simulink model "Partie4_Registre"  (R2026b)
settings: Solver=FixedStepDiscrete  StopTime=65*Tb  FixedStep=Tb
undefined symbols (not defined in the file): Tb
settings Model: Creator=WORLD COMPUTERS  LastModifiedBy=WORLD COMPUTERS

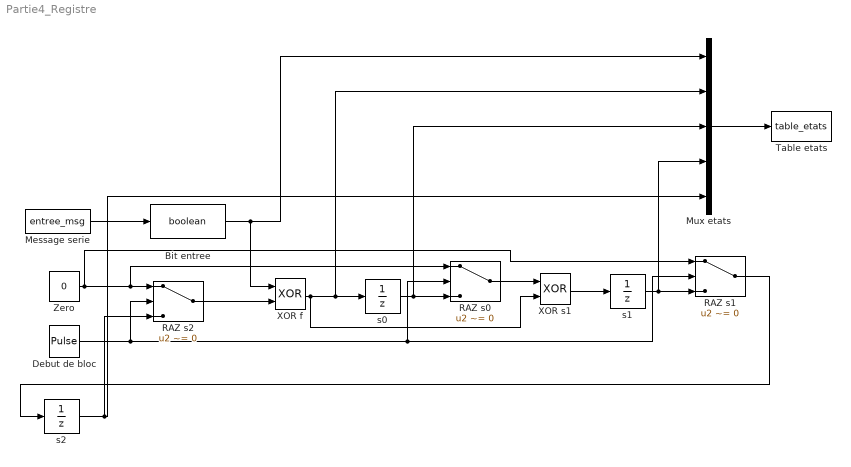
== system Partie4_Registre ==
  Bit entree : DataTypeConversion  OutDataTypeStr=boolean  SaturateOnIntegerOverflow=off  RndMeth=Floor
  Debut de bloc : DiscretePulseGenerator  Period=4  SampleTime=Tb
  Message serie : FromWorkspace  VariableName=entree_msg  SampleTime=Tb  Interpolate=off  OutputAfterFinalValue=Setting to zero
  Mux etats : Mux  Inputs=5
  RAZ s0 : Switch  Criteria=u2 ~= 0  SaturateOnIntegerOverflow=off  InputSameDT=off
  RAZ s1 : Switch  Criteria=u2 ~= 0  SaturateOnIntegerOverflow=off  InputSameDT=off
  RAZ s2 : Switch  Criteria=u2 ~= 0  SaturateOnIntegerOverflow=off  InputSameDT=off
  Table etats : ToWorkspace  VariableName=table_etats  SampleTime=-1
  XOR f : Logic  Operator=XOR  AllPortsSameDT=off  OutDataTypeStr=boolean
  XOR s1 : Logic  Operator=XOR  AllPortsSameDT=off  OutDataTypeStr=boolean
  Zero : Constant  Value=0  OutDataTypeStr=boolean
  s0 : UnitDelay  SampleTime=Tb
  s1 : UnitDelay  SampleTime=Tb
  s2 : UnitDelay  SampleTime=Tb
  wires:
  Message serie/1 -> Bit entree/1
  Debut de bloc/1 -> RAZ s0/2, RAZ s1/2, RAZ s2/2
  s0/1 -> Mux etats/3, RAZ s0/3
  Bit entree/1 -> Mux etats/1, XOR f/1
  Zero/1 -> RAZ s0/1, RAZ s2/1, RAZ s1/1
  RAZ s1/1 -> s2/1
  RAZ s0/1 -> XOR s1/1
  RAZ s2/1 -> XOR f/2
  s1/1 -> RAZ s1/3, Mux etats/4
  s2/1 -> Mux etats/5, RAZ s2/3
  XOR f/1 -> Mux etats/2, s0/1, XOR s1/2
  Mux etats/1 -> Table etats/1
  XOR s1/1 -> s1/1
